simulink model "IEEE33_TR_TEMPORAL_RECOGNIZABILITY_MASTER"  (R2026b)
settings: Solver=ode23t  StopTime=0.2  MaxStep=1e-5
undefined symbols (not defined in the file): Three_PhaseBreaker_class, Three_PhaseSeriesRLCLoad_class, Three_PhaseSource_class, Three_PhaseV_IMeasuremen_class
libraries: ee_lib x146, nesl_utility x106, fl_lib x33, eeRmsMeasurement x2
(part 7 of 7)

== system IEEE33_TR_TEMPORAL_RECOGNIZABILITY_MASTER/Bus_7/VI Recorder10 ==
  Vrec : Inport
  Irec : Inport  Port=2
  tag scope: I6to7=global, V6to7=global
  wires:
  Vrec/1 -> [V6to7]
  Irec/1 -> [I6to7]

== system IEEE33_TR_TEMPORAL_RECOGNIZABILITY_MASTER/Bus_8/Bus Load 8 ==
  Electrical Reference : fl_lib/Electrical/Electrical Elements/Electrical Reference
  Wye-Connected Load : ee_lib/Passive/RLC Assemblies/Wye-Connected Load  port_option=ee.enum.threePhasePort.expanded  parameterization=2  component_structure=4  component_structure_PQ=4  R=1 Ohm  L=0.001 H  C=1e-6 F  VRated=11918.2126 V  FRated=60 Hz  P=200000 W  Qpos=100000 V*A  Qneg=Three_PhaseSeriesRLCLoad_class(0).objParamMappingDerived.NewDerivedParam.Qneg V*A  R_parasitic=1e-6 Ohm  G_parasitic=1e-6 1/Ohm  R_parasitic_PQ=1e-6 Ohm  G_parasitic_PQ=1e-6 1/Ohm  Vmag0=11918.2126 V  Vang0=0 deg  Freq0=60 Hz  IL_specify=on  IL_priority=High  IL=[ 0 0 0 ] A  IL_nominal_specify=off  IL_nominal_value=1  IL_nominal_unit=A  VC_specify=on  VC_priority=High  VC=[ 0 0 0 ] V  VC_nominal_specify=off  VC_nominal_value=1  VC_nominal_unit=V
  A : PMIOPort  Side=Left
  B : PMIOPort  Port=2  Side=Left
  C : PMIOPort  Port=3  Side=Left
  connections:
  Electrical Reference/LConn1 -- Wye-Connected Load/RConn1
  Wye-Connected Load/LConn3 -- C/RConn1
  Wye-Connected Load/LConn1 -- A/RConn1
  Wye-Connected Load/LConn2 -- B/RConn1

== system IEEE33_TR_TEMPORAL_RECOGNIZABILITY_MASTER/Bus_8/Bus_8 ==
  Current and Voltage Sensor (Three-Phase) : ee_lib/Sensors & Transducers/Current and Voltage Sensor (Three-Phase)  port_option=ee.enum.threePhasePort.expanded  vMeasurementType=1  outputUnit=2  SRated=100000000 V*A  VRated=500000 V  I_specify=off  I_priority=None  I=[ 0 0 0 ] A  I_nominal_specify=off  I_nominal_value=1  I_nominal_unit=A  V_specify=off  V_priority=None  V=[ 0 0 0 ] V  V_nominal_specify=off  V_nominal_value=1  V_nominal_unit=V
  Igain : Gain  Gain=Three_PhaseV_IMeasuremen_class('phase-to-phase','yes','off','off','off',100000000,500000).objParamMappingDerived.NewDerivedParam.IG
  PS-Simulink Converter : nesl_utility/PS-Simulink Converter  PhysicalDomain=network_engine_domain  SubClassName=ps_output  LeftPortType=input  RightPortType=output  PseudoPeriodic=off  Frequencies=[]  VectorFormat=1-D array  Unit=1  AffineConversion=off
  PS-Simulink Converter1 : nesl_utility/PS-Simulink Converter  PhysicalDomain=network_engine_domain  SubClassName=ps_output  LeftPortType=input  RightPortType=output  PseudoPeriodic=off  Frequencies=[]  VectorFormat=1-D array  Unit=1  AffineConversion=off
  Vgain : Gain  Gain=Three_PhaseV_IMeasuremen_class('phase-to-phase','yes','off','off','off',100000000,500000).objParamMappingDerived.NewDerivedParam.VG
  A : PMIOPort  Side=Left
  B : PMIOPort  Port=2  Side=Left
  C : PMIOPort  Port=3  Side=Left
  a : PMIOPort  Port=4  Side=Right
  b : PMIOPort  Port=5  Side=Right
  c : PMIOPort  Port=6  Side=Right
  Vabc : Outport  VectorParamsAs1DForOutWhenUnconnected=off
  Iabc : Outport  Port=2  VectorParamsAs1DForOutWhenUnconnected=off
  wires:
  Igain/1 -> Iabc/1
  Vgain/1 -> Vabc/1
  PS-Simulink Converter1/1 -> Igain/1
  PS-Simulink Converter/1 -> Vgain/1
  connections:
  Current and Voltage Sensor (Three-Phase)/RConn1 -- PS-Simulink Converter/LConn1
  Current and Voltage Sensor (Three-Phase)/RConn2 -- PS-Simulink Converter1/LConn1
  Current and Voltage Sensor (Three-Phase)/RConn5 -- c/RConn1
  Current and Voltage Sensor (Three-Phase)/RConn4 -- b/RConn1
  Current and Voltage Sensor (Three-Phase)/RConn3 -- a/RConn1
  Current and Voltage Sensor (Three-Phase)/LConn3 -- C/RConn1
  Current and Voltage Sensor (Three-Phase)/LConn1 -- A/RConn1
  Current and Voltage Sensor (Three-Phase)/LConn2 -- B/RConn1

== system IEEE33_TR_TEMPORAL_RECOGNIZABILITY_MASTER/Bus_8/CB3-2 ==
  com : Inport
  Add : Sum
  Circuit Breaker : ee_lib/Switches & Breakers/Circuit Breaker (Three-Phase)  port_option=ee.enum.threePhasePort.expanded  control_port_option=ee.enum.controlport.ps  R_closed=0.01 Ohm  G_open=Three_PhaseBreaker_class('open',1000000,Inf,[0.0166666666666667 0.0833333333333333],'on').objParamMappingDerived.NewDerivedParam.G_open 1/Ohm  threshold=0.5 V  breaker_behavior=ee.enum.switches.breakerBehavior.zeroCrossingEnable  i_th=1e-8 A
  Data Type Conversion : DataTypeConversion  OutDataTypeStr=double  SaturateOnIntegerOverflow=off  RndMeth=Floor
  NOT : Logic  Operator=NOT  IconShape=distinctive  AllPortsSameDT=off  OutDataTypeStr=boolean
  Simulink-PS Converter : nesl_utility/Simulink-PS Converter  PhysicalDomain=network_engine_domain  SubClassName=ps_input  LeftPortType=input  RightPortType=output  PseudoPeriodic=off  Frequencies=[]  NoiseDistribution=none  NoiseParameters=[]  Unit=1  AffineConversion=off  FilteringAndDerivatives=provide  SimscapeFilterOrder=1  InputFilterTimeConstant=0.001  UdotUserProvided=0
  Step : Step  Time=1e-6  InitialValue=Three_PhaseBreaker_class('open',1000000,Inf,[0.0166666666666667 0.0833333333333333],'on').objParamMappingDerived.NewDerivedParam.StepInitialValue  FinalValue=0  SampleTime=0
  A : PMIOPort  Side=Left
  B : PMIOPort  Port=2  Side=Left
  C : PMIOPort  Port=3  Side=Left
  a : PMIOPort  Port=4  Side=Right
  b : PMIOPort  Port=5  Side=Right
  c : PMIOPort  Port=6  Side=Right
  wires:
  com/1 -> Add/1
  Add/1 -> NOT/1
  Step/1 -> Add/2
  Data Type Conversion/1 -> Simulink-PS Converter/1
  NOT/1 -> Data Type Conversion/1
  connections:
  Circuit Breaker/LConn1 -- Simulink-PS Converter/RConn1
  c/RConn1 -- Circuit Breaker/RConn3
  b/RConn1 -- Circuit Breaker/RConn2
  a/RConn1 -- Circuit Breaker/RConn1
  Circuit Breaker/LConn4 -- C/RConn1
  Circuit Breaker/LConn3 -- B/RConn1
  Circuit Breaker/LConn2 -- A/RConn1

== system IEEE33_TR_TEMPORAL_RECOGNIZABILITY_MASTER/Bus_8/VI Recorder11 ==
  Vrec : Inport
  Irec : Inport  Port=2
  tag scope: I7to8=global, V7to8=global
  wires:
  Vrec/1 -> [V7to8]
  Irec/1 -> [I7to8]

== system IEEE33_TR_TEMPORAL_RECOGNIZABILITY_MASTER/Bus_9/Bus Load 9 ==
  Electrical Reference : fl_lib/Electrical/Electrical Elements/Electrical Reference
  Wye-Connected Load : ee_lib/Passive/RLC Assemblies/Wye-Connected Load  port_option=ee.enum.threePhasePort.expanded  parameterization=2  component_structure=4  component_structure_PQ=4  R=1 Ohm  L=0.001 H  C=1e-6 F  VRated=11838.9737 V  FRated=60 Hz  P=60000 W  Qpos=20000 V*A  Qneg=Three_PhaseSeriesRLCLoad_class(0).objParamMappingDerived.NewDerivedParam.Qneg V*A  R_parasitic=1e-6 Ohm  G_parasitic=1e-6 1/Ohm  R_parasitic_PQ=1e-6 Ohm  G_parasitic_PQ=1e-6 1/Ohm  Vmag0=11838.9737 V  Vang0=0 deg  Freq0=60 Hz  IL_specify=on  IL_priority=High  IL=[ 0 0 0 ] A  IL_nominal_specify=off  IL_nominal_value=1  IL_nominal_unit=A  VC_specify=on  VC_priority=High  VC=[ 0 0 0 ] V  VC_nominal_specify=off  VC_nominal_value=1  VC_nominal_unit=V
  A : PMIOPort  Side=Left
  B : PMIOPort  Port=2  Side=Left
  C : PMIOPort  Port=3  Side=Left
  connections:
  Electrical Reference/LConn1 -- Wye-Connected Load/RConn1
  Wye-Connected Load/LConn3 -- C/RConn1
  Wye-Connected Load/LConn1 -- A/RConn1
  Wye-Connected Load/LConn2 -- B/RConn1

== system IEEE33_TR_TEMPORAL_RECOGNIZABILITY_MASTER/Bus_9/Bus_9 ==
  Current and Voltage Sensor (Three-Phase) : ee_lib/Sensors & Transducers/Current and Voltage Sensor (Three-Phase)  port_option=ee.enum.threePhasePort.expanded  vMeasurementType=1  outputUnit=2  SRated=100000000 V*A  VRated=500000 V  I_specify=off  I_priority=None  I=[ 0 0 0 ] A  I_nominal_specify=off  I_nominal_value=1  I_nominal_unit=A  V_specify=off  V_priority=None  V=[ 0 0 0 ] V  V_nominal_specify=off  V_nominal_value=1  V_nominal_unit=V
  Igain : Gain  Gain=Three_PhaseV_IMeasuremen_class('phase-to-phase','yes','off','off','off',100000000,500000).objParamMappingDerived.NewDerivedParam.IG
  PS-Simulink Converter : nesl_utility/PS-Simulink Converter  PhysicalDomain=network_engine_domain  SubClassName=ps_output  LeftPortType=input  RightPortType=output  PseudoPeriodic=off  Frequencies=[]  VectorFormat=1-D array  Unit=1  AffineConversion=off
  PS-Simulink Converter1 : nesl_utility/PS-Simulink Converter  PhysicalDomain=network_engine_domain  SubClassName=ps_output  LeftPortType=input  RightPortType=output  PseudoPeriodic=off  Frequencies=[]  VectorFormat=1-D array  Unit=1  AffineConversion=off
  Vgain : Gain  Gain=Three_PhaseV_IMeasuremen_class('phase-to-phase','yes','off','off','off',100000000,500000).objParamMappingDerived.NewDerivedParam.VG
  A : PMIOPort  Side=Left
  B : PMIOPort  Port=2  Side=Left
  C : PMIOPort  Port=3  Side=Left
  a : PMIOPort  Port=4  Side=Right
  b : PMIOPort  Port=5  Side=Right
  c : PMIOPort  Port=6  Side=Right
  Vabc : Outport  VectorParamsAs1DForOutWhenUnconnected=off
  Iabc : Outport  Port=2  VectorParamsAs1DForOutWhenUnconnected=off
  wires:
  Igain/1 -> Iabc/1
  Vgain/1 -> Vabc/1
  PS-Simulink Converter1/1 -> Igain/1
  PS-Simulink Converter/1 -> Vgain/1
  connections:
  Current and Voltage Sensor (Three-Phase)/RConn1 -- PS-Simulink Converter/LConn1
  Current and Voltage Sensor (Three-Phase)/RConn2 -- PS-Simulink Converter1/LConn1
  Current and Voltage Sensor (Three-Phase)/RConn5 -- c/RConn1
  Current and Voltage Sensor (Three-Phase)/RConn4 -- b/RConn1
  Current and Voltage Sensor (Three-Phase)/RConn3 -- a/RConn1
  Current and Voltage Sensor (Three-Phase)/LConn3 -- C/RConn1
  Current and Voltage Sensor (Three-Phase)/LConn1 -- A/RConn1
  Current and Voltage Sensor (Three-Phase)/LConn2 -- B/RConn1

== system IEEE33_TR_TEMPORAL_RECOGNIZABILITY_MASTER/Bus_9/CB3-1 ==
  com : Inport
  Add : Sum
  Circuit Breaker : ee_lib/Switches & Breakers/Circuit Breaker (Three-Phase)  port_option=ee.enum.threePhasePort.expanded  control_port_option=ee.enum.controlport.ps  R_closed=0.01 Ohm  G_open=Three_PhaseBreaker_class('open',1000000,Inf,[0.0166666666666667 0.0833333333333333],'on').objParamMappingDerived.NewDerivedParam.G_open 1/Ohm  threshold=0.5 V  breaker_behavior=ee.enum.switches.breakerBehavior.zeroCrossingEnable  i_th=1e-8 A
  Data Type Conversion : DataTypeConversion  OutDataTypeStr=double  SaturateOnIntegerOverflow=off  RndMeth=Floor
  NOT : Logic  Operator=NOT  IconShape=distinctive  AllPortsSameDT=off  OutDataTypeStr=boolean
  Simulink-PS Converter : nesl_utility/Simulink-PS Converter  PhysicalDomain=network_engine_domain  SubClassName=ps_input  LeftPortType=input  RightPortType=output  PseudoPeriodic=off  Frequencies=[]  NoiseDistribution=none  NoiseParameters=[]  Unit=1  AffineConversion=off  FilteringAndDerivatives=provide  SimscapeFilterOrder=1  InputFilterTimeConstant=0.001  UdotUserProvided=0
  Step : Step  Time=1e-6  InitialValue=Three_PhaseBreaker_class('open',1000000,Inf,[0.0166666666666667 0.0833333333333333],'on').objParamMappingDerived.NewDerivedParam.StepInitialValue  FinalValue=0  SampleTime=0
  A : PMIOPort  Side=Left
  B : PMIOPort  Port=2  Side=Left
  C : PMIOPort  Port=3  Side=Left
  a : PMIOPort  Port=4  Side=Right
  b : PMIOPort  Port=5  Side=Right
  c : PMIOPort  Port=6  Side=Right
  wires:
  com/1 -> Add/1
  Add/1 -> NOT/1
  Step/1 -> Add/2
  Data Type Conversion/1 -> Simulink-PS Converter/1
  NOT/1 -> Data Type Conversion/1
  connections:
  Circuit Breaker/LConn1 -- Simulink-PS Converter/RConn1
  c/RConn1 -- Circuit Breaker/RConn3
  b/RConn1 -- Circuit Breaker/RConn2
  a/RConn1 -- Circuit Breaker/RConn1
  Circuit Breaker/LConn4 -- C/RConn1
  Circuit Breaker/LConn3 -- B/RConn1
  Circuit Breaker/LConn2 -- A/RConn1

== system IEEE33_TR_TEMPORAL_RECOGNIZABILITY_MASTER/Bus_9/CB3-2 ==
  com : Inport
  Add : Sum
  Circuit Breaker : ee_lib/Switches & Breakers/Circuit Breaker (Three-Phase)  port_option=ee.enum.threePhasePort.expanded  control_port_option=ee.enum.controlport.ps  R_closed=0.01 Ohm  G_open=Three_PhaseBreaker_class('open',1000000,Inf,[0.0166666666666667 0.0833333333333333],'on').objParamMappingDerived.NewDerivedParam.G_open 1/Ohm  threshold=0.5 V  breaker_behavior=ee.enum.switches.breakerBehavior.zeroCrossingEnable  i_th=1e-8 A
  Data Type Conversion : DataTypeConversion  OutDataTypeStr=double  SaturateOnIntegerOverflow=off  RndMeth=Floor
  NOT : Logic  Operator=NOT  IconShape=distinctive  AllPortsSameDT=off  OutDataTypeStr=boolean
  Simulink-PS Converter : nesl_utility/Simulink-PS Converter  PhysicalDomain=network_engine_domain  SubClassName=ps_input  LeftPortType=input  RightPortType=output  PseudoPeriodic=off  Frequencies=[]  NoiseDistribution=none  NoiseParameters=[]  Unit=1  AffineConversion=off  FilteringAndDerivatives=provide  SimscapeFilterOrder=1  InputFilterTimeConstant=0.001  UdotUserProvided=0
  Step : Step  Time=1e-6  InitialValue=Three_PhaseBreaker_class('open',1000000,Inf,[0.0166666666666667 0.0833333333333333],'on').objParamMappingDerived.NewDerivedParam.StepInitialValue  FinalValue=0  SampleTime=0
  A : PMIOPort  Side=Left
  B : PMIOPort  Port=2  Side=Left
  C : PMIOPort  Port=3  Side=Left
  a : PMIOPort  Port=4  Side=Right
  b : PMIOPort  Port=5  Side=Right
  c : PMIOPort  Port=6  Side=Right
  wires:
  com/1 -> Add/1
  Add/1 -> NOT/1
  Step/1 -> Add/2
  Data Type Conversion/1 -> Simulink-PS Converter/1
  NOT/1 -> Data Type Conversion/1
  connections:
  Circuit Breaker/LConn1 -- Simulink-PS Converter/RConn1
  c/RConn1 -- Circuit Breaker/RConn3
  b/RConn1 -- Circuit Breaker/RConn2
  a/RConn1 -- Circuit Breaker/RConn1
  Circuit Breaker/LConn4 -- C/RConn1
  Circuit Breaker/LConn3 -- B/RConn1
  Circuit Breaker/LConn2 -- A/RConn1

== system IEEE33_TR_TEMPORAL_RECOGNIZABILITY_MASTER/Bus_9/VI Recorder12 ==
  Vrec : Inport
  Irec : Inport  Port=2
  tag scope: I8to9=global, V8to9=global
  wires:
  Vrec/1 -> [V8to9]
  Irec/1 -> [I8to9]
